simulink model "OSWEC"  (R2015b)
settings: Solver=ode4  StartTime=0  StopTime=400  FixedStep=0.1  RelTol=1e-3
undefined symbols (not defined in the file or in its folder): body, constraint, pto
libraries: WECSim_Lib x5
settings Model: Creator=mlawson  LastModifiedBy=kmruehl
settings SolverCC: AlgebraicLoopSolver=LineSearch
settings DataIOCC: LimitDataPoints=off  SaveFormat=Array  SaveOutput=off  SaveTime=off
settings DebuggingCC: UnderspecifiedInitializationDetection=Classic  MergeDetectMultiDrivingBlocksExec=none  SolverPrmCheckMsg=warning  StateNameClashWarn=warning
settings HardwareCC: ProdBitPerPointer=32  ProdLargestAtomicFloat=None  ProdIntDivRoundTo=Undefined  ProdEndianess=Unspecified  ProdWordSize=32  ProdHWDeviceType=32-bit Generic
settings GRTTargetCC: GeneratePreprocessorConditionals=Disable all
settings ConfigComp: CovModelRefEnable=Off  CovSFcnEnable=off
settings ExplorerConfigSet: InternalSimMechanicsExplorerSettings="<ExplorerConfiguration><canonicalview>default</canonicalview><TilePanel><TileInfo><Tiles Columns=\"1\" Count=\"1\" Rows=\"1\"><Column Left=\"2\" Weight=\"1\"/><Column Left=\"1335\"/><Row Top=\"2\" Weight=\"1\"/><Row Top=\"911\"/><Tile Height=\"1\" Width=\"1\" X=\"0\" Y=\"0\"/></Tiles></TileInfo><SceneInfo><SceneViewer><BGColor><R>0.60000002384185791</R><G>0.60000002384185791</G><B>0.60000002384185791</B></BGColor><Camera><Position><X>365.37645888990272</X><Y>-369.82486814446582</Y><Z>359.64809521743916</Z></Position><Center><X>-6.7351450971904585</X><Y>2.2867358426280204</Y><Z>-12.463508769654169</Z></Center><Up><X>-0.40824829046386307</X><Y>0.40824829046386307</Y><Z>0.81649658092772615</Z></Up><Left>-57.820127362122818</Left><Right>57.820127362122818</Right><Bottom>-38.308817187253304</Bottom><Top>38.308817187253304</Top></Camera></SceneViewer></SceneInfo></TilePanel></ExplorerConfiguration>"

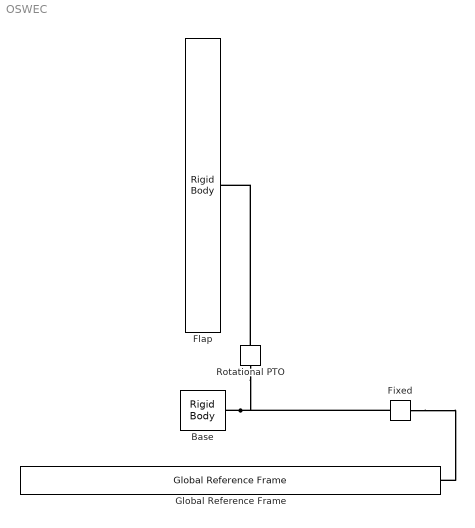
== system OSWEC ==
  Base : WECSim_Lib/Body Elements/Rigid Body  body=body(2)
      settings: AttributesFormatString=%<body>
  Fixed : WECSim_Lib/Constraints/Fixed  constraint=constraint(1)
      settings: AttributesFormatString=%<constraint>
  Flap : WECSim_Lib/Body Elements/Rigid Body  body=body(1)
      settings: AttributesFormatString=%<body>
  Global Reference Frame : WECSim_Lib/Frames/Global Reference Frame  waves=waves  simu=simu
  Rotational PTO : WECSim_Lib/PTOs/Rotational PTO  pto=pto(1)
      settings: AttributesFormatString=%<pto>
  connections:
  Fixed/LConn1 -- Global Reference Frame/RConn1
  Base/RConn1 -- Fixed/RConn1 -- Rotational PTO/LConn1
  Rotational PTO/RConn1 -- Flap/RConn1
